simulink model "BLDC_SVM"  (R2023b)
settings: Solver=FixedStepDiscrete  StartTime=0.0  StopTime=10  FixedStep=1e-5  RelTol=1e-5
undefined symbols (not defined in the file): DiscIntNeverNeededParam
libraries: slpidlib x3, simulink x3, spsCurrentMeasurementLib x2, spsAlphaBetaZerotodq0Lib x1, spsDCVoltageSourceLib x1, spsPermanentMagnetSynchronousMachineLib x1, spsSVPWMGenerator2LevelLib x1, spsUniversalBridgeLib x1, spsVoltageMeasurementLib x1, spsabctoAlphaBetaZeroLib x1, spsdq0toAlphaBetaZeroLib x1, sps_lib x1
settings Model: Creator=84339  LastModifiedBy=84339
settings OptimizationCC: DefaultParameterBehavior=Inlined  EnhancedBackFolding=on  PassReuseOutputArgsAs=Individual arguments  ZeroExternalMemoryAtStartup=off  ZeroInternalMemoryAtStartup=off  OptimizeBlockOrder=speed  DifferentSizesBufferReuse=on  OptimizationCustomize=off  EfficientTunableParamExpr=on
settings DebuggingCC: ParameterTunabilityLossMsg=error
settings SFSimCC: MATLABDynamicMemAlloc=off
settings RTWCC: Description=Embedded Coder  SystemTargetFile=ert.tlc  GenCodeOnly=on  TemplateMakefile=ert_default_tmf
settings CodeAppCC: ForceParamTrailComments=on  IgnoreCustomStorageClasses=off  OperatorAnnotations=on  SimulinkDataObjDesc=on  SFDataObjDesc=on  InsertBlockDesc=on
settings ERTTargetCC: TargetLangStandard=C99 (ISO)  GenerateSampleERTMain=on  SupportContinuousTime=on  InlinedParameterPlacement=NonHierarchical  ERTCustomFileTemplate=example_file_process.tlc

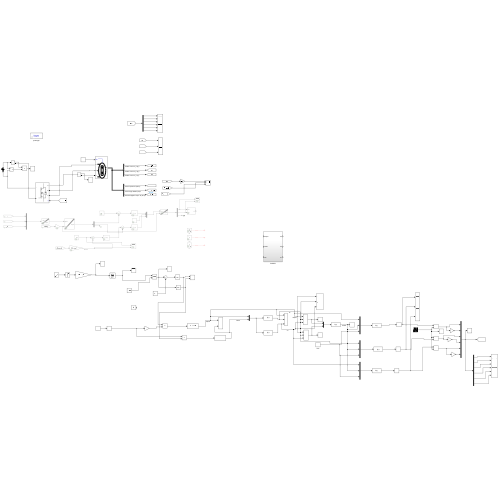
[thumbnail: Simulink's stored preview of the top-level diagram]
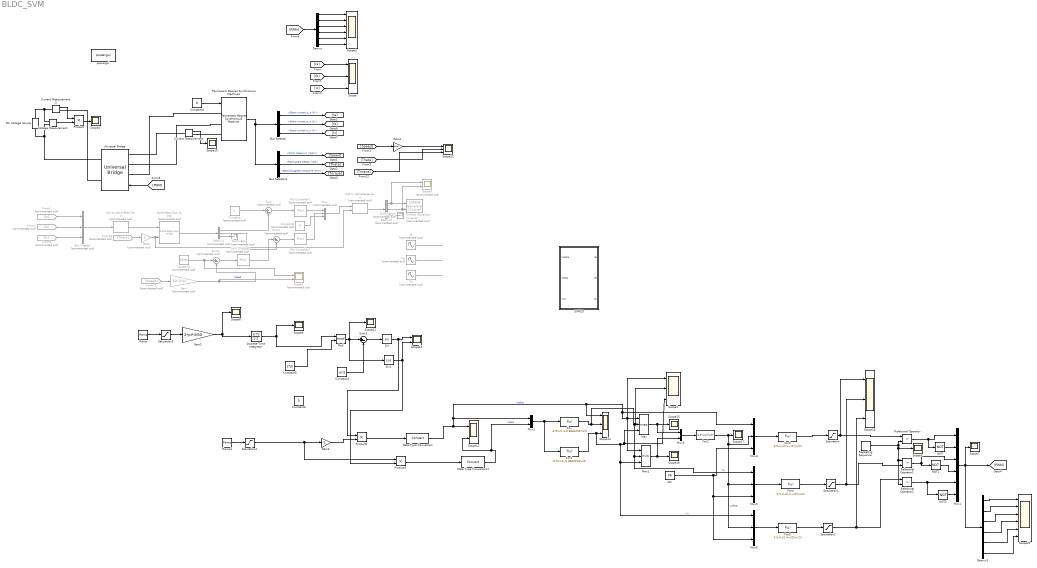
== system BLDC_SVM ==
  Alpha-Beta-Zero to dq0 : spsAlphaBetaZerotodq0Lib/Alpha-Beta-Zero to dq0  Commented=on  Alignment=90 degrees behind phase A axis
  Bus Creator : BusCreator  Commented=on  Inputs=3
  Bus Selector : BusSelector  OutputSignals=Stator current is_a (A),Stator current is_b (A),Stator current is_c (A)
  Bus Selector1 : BusSelector  OutputSignals=Rotor speed wm (rad/s),Rotor angle thetam (rad),Electromagnetic torque Te (N*m)
  Constant : Constant  Commented=on  Value=0
  Constant1 : Constant  Commented=on  Value=2500
  Constant2 : Constant  Commented=on  Value=0
  Constant3 : Constant  Value=pi/2  OutDataTypeStr=single
  Constant4 : Constant  Value=0
  Constant5 : Constant  Value=2*pi  OutDataTypeStr=single
  Constant6 : Constant  Value=0
  Current Measurement : spsCurrentMeasurementLib/Current Measurement  PhasorSimulation=off  OutputType=Complex  PSBequivalent=0
  Current Measurement3 : spsCurrentMeasurementLib/Current Measurement  PhasorSimulation=off  OutputType=Complex  PSBequivalent=0
  DC Voltage Source : spsDCVoltageSourceLib/DC Voltage Source  Amplitude=36  Measurements=None
  Data Type Conversion : DataTypeConversion  SaturateOnIntegerOverflow=off  RndMeth=Floor
  Data Type Conversion1 : DataTypeConversion  SaturateOnIntegerOverflow=off  RndMeth=Floor
  Demux : Demux  Outputs=6
  Demux1 : Demux  Commented=on  Outputs=3
  Demux2 : Demux  Commented=on  Outputs=3
  Demux3 : Demux  Outputs=6
  Discrete-Time Integrator : DiscreteIntegrator  SampleTime=1e-4  ICPrevOutput=DiscIntNeverNeededParam  ICPrevScaledInput=DiscIntNeverNeededParam
  Fcn : Fcn  Expr=-0.5*u(1)+0.8660254*u(2)
  Fcn1 : Fcn  Expr=-0.5*u(1)-0.8660254*u(2)
  Fcn2 : Fcn  Expr=-0.5*(u(1)+u(2))
  Fcn3 : Fcn  Expr=0.5+(u(1)+u(2))/u(3)
  Fcn4 : Fcn  Expr=0.5+(u(1)+u(2))/u(3)
  Fcn5 : Fcn  Expr=0.5+(u(1)+u(2))/u(3)
  From10 : From  Commented=on  GotoTag=Theta
  From11 : From  Commented=on  GotoTag=Speed
  From6 : From  Commented=on  GotoTag=Ia
  From7 : From  Commented=on  GotoTag=Ib
  From8 : From  Commented=on  GotoTag=Ic
  Gain : Gain  Commented=on  Gain=60/(2*pi)
  Gain1 : Gain  Commented=on  Gain=4
  Gain2 : Gain  Gain=2*pi*4/60  OutDataTypeStr=single
  Gain3 : Gain  Gain=-1
  Gain4 : Gain  Gain=30/pi
  Max : MinMax  Function=max  Inputs=3
  Max1 : MinMax  Inputs=3
  Mod : Math  Operator=mod
  Mux : Mux  Commented=on  Inputs=3
  Mux1 : Mux  Inputs=6
  Mux2 : Mux  Inputs=2
  Mux3 : Mux  Inputs=2
  Mux4 : Mux  Inputs=3
  Mux5 : Mux  Inputs=3
  Mux6 : Mux  Inputs=3
  NOT : Logic  Operator=NOT  IconShape=distinctive  AllPortsSameDT=off  OutDataTypeStr=boolean
  NOT1 : Logic  Operator=NOT  IconShape=distinctive  AllPortsSameDT=off  OutDataTypeStr=boolean
  NOT2 : Logic  Operator=NOT  IconShape=distinctive  AllPortsSameDT=off  OutDataTypeStr=boolean
  PID Controller : slpidlib/PID Controller  Commented=on  Controller=PI  Form=Parallel  TimeDomain=Discrete-time  UseExternalTs=off  SampleTime=1e-5  IntegratorMethod=Forward Euler  FilterMethod=Forward Euler  ControllerParametersSource=internal  P=0.1  I=0.01  UseKiTs=off  D=0  N=100  UseFilter=on  TunerSelectOption=Transfer Function Based (PID Tuner App)  InitialConditionSource=internal  InitialConditionForIntegrator=0  InitialConditionForFilter=0  DifferentiatorICPrevScaledInput=0  ExternalReset=none  TrackingMode=off  Kt=1  LimitOutput=off  SatLimitsSource=internal  UpperSaturationLimit=inf  LowerSaturationLimit=-inf  LinearizeAsGain=on  AntiWindupMode=none  Kb=1  LimitIntegrator=off  UpperIntegratorSaturationLimit=inf  LowerIntegratorSaturationLimit=-inf  POutMin=[]  POutMax=[]  IOutMin=[]  IOutMax=[]  DOutMin=[]  DOutMax=[]  NOutMin=[]  NOutMax=[]  SumOutMin=[]  SumOutMax=[]  SaturationOutMin=[]  SaturationOutMax=[]  PParamMin=[]  PParamMax=[]  IParamMin=[]  IParamMax=[]  DParamMin=[]  DParamMax=[]  NParamMin=[]  NParamMax=[]  KbParamMin=[]  KbParamMax=[]  KtParamMin=[]  KtParamMax=[]  KbOutMin=[]  KbOutMax=[]  KtOutMin=[]  KtOutMax=[]  IntegratorOutMin=[]  IntegratorOutMax=[]  FilterOutMin=[]  FilterOutMax=[]  SumI1OutMin=[]  SumI1OutMax=[]  SumI2OutMin=[]  SumI2OutMax=[]  SumI3OutMin=[]  SumI3OutMax=[]  SumI4OutMin=[]  SumI4OutMax=[]  SumDOutMin=[]  SumDOutMax=[]  DifferentiatorOutMin=[]  DifferentiatorOutMax=[]  FilterDiffOutCoefMin=[]  FilterDiffOutCoefMax=[]  ReciprocalOutMin=[]  ReciprocalOutMax=[]  SumDenOutMin=[]  SumDenOutMax=[]  SumNumOutMin=[]  SumNumOutMax=[]  DivideOutMin=[]  DivideOutMax=[]  UdiffTsProdOutMin=[]  UdiffTsProdOutMax=[]  NTsProdOutMin=[]  NTsProdOutMax=[]  UintegralTsProdOutMin=[]  UintegralTsProdOutMax=[]  UngainTsProdOutMin=[]  UngainTsProdOutMax=[]  ClampingZeroOutDataTypeStr=Inherit: Inherit via back propagation  ClampingZeroOutMin=[]  ClampingZeroOutMax=[]  FilterDenConstantOutDataTypeStr=Inherit: Inherit via back propagation  FilterDenConstantOutMin=[]  FilterDenConstantOutMax=[]  PCopyOutDataTypeStr=Inherit: Inherit via back propagation  PCopyOutMin=[]  PCopyOutMax=[]  NCopyOutDataTypeStr=Inherit: Inherit via back propagation  NCopyOutMin=[]  NCopyOutMax=[]  IntegratorContinuousStateAttributes=''  IntegratorStateMustResolveToSignalObject=off  IntegratorRTWStateStorageClass=Auto  FilterContinuousStateAttributes=''  FilterStateMustResolveToSignalObject=off  FilterRTWStateStorageClass=Auto  ParallelPVariant=InternalParameters  IdealPVariant=Disabled  IVariant=InternalParameters  DVariant=Disabled  IntegratorVariant=Discrete  SatVariant=Disabled  AWVariant=Passthrough  PCopyVariant=Disabled  TRVariant=Disabled  FdbkBlocksVariant=Forward  IdealPFdbkVariant=Disabled  SatFdbkVariant=Disabled  DerivativeFilterVariant=Disabled  NVariant=Disabled  NCopyVariant=Disabled_SignalSpec  FilterICVariant=Disabled  IntegratorICVariant=InternalICs  ExternalResetVariant=Disabled  TRSumVariant=Passthrough  SumFdbkVariant=Disabled  SumVariant=Sum_PI  TsampFilterVariant=InternalTs  TsampNgainVariant=Passthrough  TsampIntegralVariant=Disabled_SignalSpec  ExternalSaturationOutDataTypeStr=Inherit: Same as second input
  PID Controller1 : slpidlib/PID Controller  Commented=on  Controller=PI  Form=Parallel  TimeDomain=Discrete-time  UseExternalTs=off  SampleTime=1e-5  IntegratorMethod=Forward Euler  FilterMethod=Forward Euler  ControllerParametersSource=internal  P=1  I=0.01  UseKiTs=off  D=0  N=100  UseFilter=on  TunerSelectOption=Transfer Function Based (PID Tuner App)  InitialConditionSource=internal  InitialConditionForIntegrator=0  InitialConditionForFilter=0  DifferentiatorICPrevScaledInput=0  ExternalReset=none  TrackingMode=off  Kt=1  LimitOutput=off  SatLimitsSource=internal  UpperSaturationLimit=inf  LowerSaturationLimit=-inf  LinearizeAsGain=on  AntiWindupMode=none  Kb=1  LimitIntegrator=off  UpperIntegratorSaturationLimit=inf  LowerIntegratorSaturationLimit=-inf  POutMin=[]  POutMax=[]  IOutMin=[]  IOutMax=[]  DOutMin=[]  DOutMax=[]  NOutMin=[]  NOutMax=[]  SumOutMin=[]  SumOutMax=[]  SaturationOutMin=[]  SaturationOutMax=[]  PParamMin=[]  PParamMax=[]  IParamMin=[]  IParamMax=[]  DParamMin=[]  DParamMax=[]  NParamMin=[]  NParamMax=[]  KbParamMin=[]  KbParamMax=[]  KtParamMin=[]  KtParamMax=[]  KbOutMin=[]  KbOutMax=[]  KtOutMin=[]  KtOutMax=[]  IntegratorOutMin=[]  IntegratorOutMax=[]  FilterOutMin=[]  FilterOutMax=[]  SumI1OutMin=[]  SumI1OutMax=[]  SumI2OutMin=[]  SumI2OutMax=[]  SumI3OutMin=[]  SumI3OutMax=[]  SumI4OutMin=[]  SumI4OutMax=[]  SumDOutMin=[]  SumDOutMax=[]  DifferentiatorOutMin=[]  DifferentiatorOutMax=[]  FilterDiffOutCoefMin=[]  FilterDiffOutCoefMax=[]  ReciprocalOutMin=[]  ReciprocalOutMax=[]  SumDenOutMin=[]  SumDenOutMax=[]  SumNumOutMin=[]  SumNumOutMax=[]  DivideOutMin=[]  DivideOutMax=[]  UdiffTsProdOutMin=[]  UdiffTsProdOutMax=[]  NTsProdOutMin=[]  NTsProdOutMax=[]  UintegralTsProdOutMin=[]  UintegralTsProdOutMax=[]  UngainTsProdOutMin=[]  UngainTsProdOutMax=[]  ClampingZeroOutDataTypeStr=Inherit: Inherit via back propagation  ClampingZeroOutMin=[]  ClampingZeroOutMax=[]  FilterDenConstantOutDataTypeStr=Inherit: Inherit via back propagation  FilterDenConstantOutMin=[]  FilterDenConstantOutMax=[]  PCopyOutDataTypeStr=Inherit: Inherit via back propagation  PCopyOutMin=[]  PCopyOutMax=[]  NCopyOutDataTypeStr=Inherit: Inherit via back propagation  NCopyOutMin=[]  NCopyOutMax=[]  IntegratorContinuousStateAttributes=''  IntegratorStateMustResolveToSignalObject=off  IntegratorRTWStateStorageClass=Auto  FilterContinuousStateAttributes=''  FilterStateMustResolveToSignalObject=off  FilterRTWStateStorageClass=Auto  ParallelPVariant=InternalParameters  IdealPVariant=Disabled  IVariant=InternalParameters  DVariant=Disabled  IntegratorVariant=Discrete  SatVariant=Disabled  AWVariant=Passthrough  PCopyVariant=Disabled  TRVariant=Disabled  FdbkBlocksVariant=Forward  IdealPFdbkVariant=Disabled  SatFdbkVariant=Disabled  DerivativeFilterVariant=Disabled  NVariant=Disabled  NCopyVariant=Disabled_SignalSpec  FilterICVariant=Disabled  IntegratorICVariant=InternalICs  ExternalResetVariant=Disabled  TRSumVariant=Passthrough  SumFdbkVariant=Disabled  SumVariant=Sum_PI  TsampFilterVariant=InternalTs  TsampNgainVariant=Passthrough  TsampIntegralVariant=Disabled_SignalSpec  ExternalSaturationOutDataTypeStr=Inherit: Same as second input
  PID Controller2 : slpidlib/PID Controller  Commented=on  Controller=PI  Form=Parallel  TimeDomain=Discrete-time  UseExternalTs=off  SampleTime=1e-5  IntegratorMethod=Forward Euler  FilterMethod=Forward Euler  ControllerParametersSource=internal  P=1  I=0.01  UseKiTs=off  D=0  N=100  UseFilter=on  TunerSelectOption=Transfer Function Based (PID Tuner App)  InitialConditionSource=internal  InitialConditionForIntegrator=0  InitialConditionForFilter=0  DifferentiatorICPrevScaledInput=0  ExternalReset=none  TrackingMode=off  Kt=1  LimitOutput=off  SatLimitsSource=internal  UpperSaturationLimit=inf  LowerSaturationLimit=-inf  LinearizeAsGain=on  AntiWindupMode=none  Kb=1  LimitIntegrator=off  UpperIntegratorSaturationLimit=inf  LowerIntegratorSaturationLimit=-inf  POutMin=[]  POutMax=[]  IOutMin=[]  IOutMax=[]  DOutMin=[]  DOutMax=[]  NOutMin=[]  NOutMax=[]  SumOutMin=[]  SumOutMax=[]  SaturationOutMin=[]  SaturationOutMax=[]  PParamMin=[]  PParamMax=[]  IParamMin=[]  IParamMax=[]  DParamMin=[]  DParamMax=[]  NParamMin=[]  NParamMax=[]  KbParamMin=[]  KbParamMax=[]  KtParamMin=[]  KtParamMax=[]  KbOutMin=[]  KbOutMax=[]  KtOutMin=[]  KtOutMax=[]  IntegratorOutMin=[]  IntegratorOutMax=[]  FilterOutMin=[]  FilterOutMax=[]  SumI1OutMin=[]  SumI1OutMax=[]  SumI2OutMin=[]  SumI2OutMax=[]  SumI3OutMin=[]  SumI3OutMax=[]  SumI4OutMin=[]  SumI4OutMax=[]  SumDOutMin=[]  SumDOutMax=[]  DifferentiatorOutMin=[]  DifferentiatorOutMax=[]  FilterDiffOutCoefMin=[]  FilterDiffOutCoefMax=[]  ReciprocalOutMin=[]  ReciprocalOutMax=[]  SumDenOutMin=[]  SumDenOutMax=[]  SumNumOutMin=[]  SumNumOutMax=[]  DivideOutMin=[]  DivideOutMax=[]  UdiffTsProdOutMin=[]  UdiffTsProdOutMax=[]  NTsProdOutMin=[]  NTsProdOutMax=[]  UintegralTsProdOutMin=[]  UintegralTsProdOutMax=[]  UngainTsProdOutMin=[]  UngainTsProdOutMax=[]  ClampingZeroOutDataTypeStr=Inherit: Inherit via back propagation  ClampingZeroOutMin=[]  ClampingZeroOutMax=[]  FilterDenConstantOutDataTypeStr=Inherit: Inherit via back propagation  FilterDenConstantOutMin=[]  FilterDenConstantOutMax=[]  PCopyOutDataTypeStr=Inherit: Inherit via back propagation  PCopyOutMin=[]  PCopyOutMax=[]  NCopyOutDataTypeStr=Inherit: Inherit via back propagation  NCopyOutMin=[]  NCopyOutMax=[]  IntegratorContinuousStateAttributes=''  IntegratorStateMustResolveToSignalObject=off  IntegratorRTWStateStorageClass=Auto  FilterContinuousStateAttributes=''  FilterStateMustResolveToSignalObject=off  FilterRTWStateStorageClass=Auto  ParallelPVariant=InternalParameters  IdealPVariant=Disabled  IVariant=InternalParameters  DVariant=Disabled  IntegratorVariant=Discrete  SatVariant=Disabled  AWVariant=Passthrough  PCopyVariant=Disabled  TRVariant=Disabled  FdbkBlocksVariant=Forward  IdealPFdbkVariant=Disabled  SatFdbkVariant=Disabled  DerivativeFilterVariant=Disabled  NVariant=Disabled  NCopyVariant=Disabled_SignalSpec  FilterICVariant=Disabled  IntegratorICVariant=InternalICs  ExternalResetVariant=Disabled  TRSumVariant=Passthrough  SumFdbkVariant=Disabled  SumVariant=Sum_PI  TsampFilterVariant=InternalTs  TsampNgainVariant=Passthrough  TsampIntegralVariant=Disabled_SignalSpec  ExternalSaturationOutDataTypeStr=Inherit: Same as second input
  Permanent Magnet Synchronous Machine1 : spsPermanentMagnetSynchronousMachineLib/Permanent Magnet Synchronous Machine  NbPhases=3  FluxDistribution=Trapezoidal  RotorType=Round  MechanicalLoad=Torque Tm  PresetModel=No  ShowDetailedParameters=on  MeasurementBus=off  Resistance=0.0485  Inductance=8.5e-3  dqInductances=[8.5e-3,8.5e-3]  La=0.000395  MachineConstant=Flux linkage established by magnets (V.s)  Flux=0.1194  VoltageCst=100.0283  TorqueCst=0.9552  Flat=120  Mechanical=[0.0027 0.0004924 4 0]  PolePairs=4  InitialConditions=[0,0, 0,0]  InitialConditions5ph=[0 0 0 0 0 0]  RefAngle=90 degrees behind phase A axis (modified Park)  IterativeDiscreteModel=Trapezoidal non iterative  TsBlock=-1  TsPowergui=0
  Product : Product
  Product2 : Product
  Product3 : Product
  Ramp : simulink/Sources/Ramp  slope=100  start=0  InitialOutput=0
  Ramp1 : simulink/Sources/Ramp  slope=100  start=0  InitialOutput=0
  Relational Operator : RelationalOperator  Operator=>  OutDataTypeStr=boolean  RndMeth=Simplest  InputSameDT=off
  Relational Operator1 : RelationalOperator  Operator=>  OutDataTypeStr=boolean  RndMeth=Simplest  InputSameDT=off
  Relational Operator2 : RelationalOperator  Operator=>  OutDataTypeStr=boolean  RndMeth=Simplest  InputSameDT=off
  Repeating Sequence : simulink/Sources/Repeating Sequence  rep_seq_t=[0 1/10000]  rep_seq_y=[0 1]
  SVM2D : Subsystem
  SVPWM Generator (2-Level) : spsSVPWMGenerator2LevelLib/SVPWM Generator (2-Level)  Commented=on  InputType=alpha-beta components  SwitchingPattern=Pattern #1  Fc=10000  ParUref=[0.8 -30 50]  Ts=1e-5
  Saturation : Saturate  UpperLimit=1  LowerLimit=0
  Saturation1 : Saturate  UpperLimit=1  LowerLimit=0
  Saturation2 : Saturate  UpperLimit=1  LowerLimit=0
  Saturation3 : Saturate  UpperLimit=300  LowerLimit=0
  Saturation4 : Saturate  UpperLimit=6  LowerLimit=0
  Scope{,1,12,14,18} (5 alike) : Scope  NumInputPorts=3
  Scope10 : Scope  NumInputPorts=2
  Scope{4,6..9,11,15..17,19} (10 alike) : Scope
  Scope13 : Scope  NumInputPorts=2
  Scope2 : Scope  Commented=on  NumInputPorts=2
  Scope20 : Scope  NumInputPorts=6
  Scope3 : Scope  NumInputPorts=6
  Scope5 : Scope  Commented=on  NumInputPorts=2
  Sin : Trigonometry
  Sin1 : Trigonometry  Operator=cos
  Sum : Sum  Commented=on  Inputs=|+-
  Sum1 : Sum  Commented=on  Inputs=|+-
  Sum2 : Sum  Commented=on  Inputs=|+-
  Sum3 : Sum  Inputs=|+-
  Terminator : Terminator  Commented=on
  Terminator1 : Terminator  Commented=on
  Universal Bridge : spsUniversalBridgeLib/Universal Bridge  Arms=3  SnubberResistance=1e5  SnubberCapacitance=inf  Device=MOSFET / Diodes  Ron=1e-3  Lon=0  ForwardVoltages="[  0  0  ]"  ForwardVoltage=0  GTOparameters=[ 10e-6 , 20e-6 ]  IGBTparameters=[ 1e-6 , 2e-6 ]  Measurements=None  Measurements_2=None  converterType=Rectifier
  Va : Sin  Commented=on  Amplitude=14*sqrt(2)  Frequency=100*pi  SampleTime=1e-5
  Vb : Sin  Commented=on  Amplitude=14*sqrt(2)  Frequency=100*pi  Phase=-2*pi/3  SampleTime=1e-5
  Vc : Sin  Commented=on  Amplitude=14*sqrt(2)  Frequency=100*pi  Phase=2*pi/3  SampleTime=1e-5
  Vdc : Constant  Value=36  OutDataTypeStr=single
  Voltage Measurement : spsVoltageMeasurementLib/Voltage Measurement  PhasorSimulation=off  OutputType=Complex  PSBequivalent=0
  abc to Alpha-Beta-Zero : spsabctoAlphaBetaZeroLib/abc to Alpha-Beta-Zero  Commented=on
  dq0 to Alpha-Beta-Zero : spsdq0toAlphaBetaZeroLib/dq0 to Alpha-Beta-Zero  Commented=on  Alignment=90 degrees behind phase A axis
  powergui : sps_lib/powergui  Priority=1  SimulationMode=Discrete  SampleTime=1e-5  frequency=60  Iterations=50  frequencyindice=0  Pbase=100e6  ErrMax=1e-4  UnitsV=kV  UnitsW=MW  buscounter=0  FunctionMessages=off  echomessages=off  EnableUseOfTLC=off  CurrentSourceSwitches=off  DisableSnubberDevices=off  DisableRonSwitches=off  DisableVfSwitches=off  DisplayEquations=off  AutomaticDiscreteSolvers=off  SolverType=Tustin/Backward Euler (TBE)  Interpol=off  ExternalGateDelay=off  methode=off  Ts=100  x0status=blocks  SPID=on  SwTol=0  HookPort=off  NonlinearTolerance=1e-4  nMaxIteration=100  ContinueOnMaxIteration=off  RestoreLinks=warning  ResistiveCurrentMeasurement=off  Frange=[0:2:500]  Ylog=off  Xlog=on  ShowGrid=off  save=off  variable=ZData  structure=0  ZoomFFT=off  StartTime=0.0  cycles=1  DisplayStyle=1  fundamental=60  FreqAxis=off  MaxFrequency=1000  frequencyindicesteady=1  RmsSteady=1  display=off
  wires:
  Permanent Magnet Synchronous Machine1/1 -> Bus Selector1/1, Bus Selector/1
  [Ia] -> Scope/1
  [Ib] -> Scope/2
  [Ic] -> Scope/3
  [PWM] -> Demux/1
  Demux/1 -> Scope3/1
  Demux/2 -> Scope3/2
  Demux/3 -> Scope3/3
  Demux/4 -> Scope3/4
  Demux/5 -> Scope3/5
  Demux/6 -> Scope3/6
  Current Measurement3/1 -> Product/1
  Voltage Measurement/1 -> Product/2
  Product/1 -> Scope4/1
  Bus Selector/1 -> [Ia]  "<Stator current is_a (A)>"
  Bus Selector/2 -> [Ib]  "<Stator current is_b (A)>"
  Bus Selector/3 -> [Ic]  "<Stator current is_c (A)>"
  From6/1 -> Bus Creator/1
  From7/1 -> Bus Creator/2
  From8/1 -> Bus Creator/3
  Bus Creator/1 -> abc to Alpha-Beta-Zero/1
  abc to Alpha-Beta-Zero/1 -> Alpha-Beta-Zero to dq0/1
  Bus Selector1/1 -> [Speed]  "<Rotor speed wm (rad/s)>"
  Bus Selector1/2 -> [Theta]  "<Rotor angle thetam (rad)>"
  From10/1 -> Gain1/1
  [PWM] -> Universal Bridge/1
  Bus Selector1/3 -> [Torque]  "<Electromagnetic torque Te (N*m)>"
  Gain1/1 -> dq0 to Alpha-Beta-Zero/2, Alpha-Beta-Zero to dq0/2
  From11/1 -> Gain/1
  Alpha-Beta-Zero to dq0/1 -> Demux1/1
  Demux1/1 -> Sum/2
  Demux1/2 -> Sum1/2
  Constant/1 -> Sum/1
  Sum2/1 -> PID Controller/1
  Gain/1 -> Scope2/2, Sum2/2  "Speed"
  Constant1/1 -> Scope2/1, Sum2/1
  PID Controller/1 -> Sum1/1
  Sum/1 -> PID Controller1/1
  Sum1/1 -> PID Controller2/1
  Demux1/3 -> Terminator/1
  PID Controller1/1 -> Mux/1
  Mux/1 -> dq0 to Alpha-Beta-Zero/1
  PID Controller2/1 -> Mux/2
  Constant2/1 -> Mux/3
  dq0 to Alpha-Beta-Zero/1 -> Demux2/1
  Demux2/3 -> Terminator1/1
  Demux2/1 -> Scope5/1, SVPWM Generator (2-Level)/1
  Demux2/2 -> Scope5/2, SVPWM Generator (2-Level)/2
  NOT/1 -> Mux1/2
  NOT1/1 -> Mux1/4
  NOT2/1 -> Mux1/6
  Mux1/1 -> Demux3/1, Scope7/1, [PWM]
  Repeating Sequence/1 -> Relational Operator2/2, Relational Operator1/1, Scope6/1, Relational Operator/2
  Saturation/1 -> Scope18/1, Relational Operator/1
  Relational Operator/1 -> NOT/1, Mux1/1
  Saturation1/1 -> Scope18/2, Relational Operator1/2
  Relational Operator1/1 -> Mux1/3, NOT1/1
  Saturation2/1 -> Scope18/3, Relational Operator2/1
  Relational Operator2/1 -> NOT2/1, Mux1/5
  Ramp/1 -> Saturation3/1
  Va/1 -> ?
  Vc/1 -> ?
  Vb/1 -> ?
  Constant5/1 -> Mod/2
  Gain2/1 -> Scope8/1, Discrete-Time Integrator/1
  Discrete-Time Integrator/1 -> Mod/1, Scope9/1
  Mod/1 -> Sum3/1, Sin1/1, Scope11/1
  Sin/1 -> Product2/1, Scope10/1
  Sin1/1 -> Product3/2, Scope10/2
  Saturation4/1 -> Product3/1, Gain3/1
  Gain3/1 -> Product2/2
  Product2/1 -> Data Type Conversion/1
  Product3/1 -> Data Type Conversion1/1
  [Speed] -> Gain4/1
  Data Type Conversion1/1 -> Scope13/2, Mux2/2  "Vbeta"
  Mux2/1 -> Fcn1/1, Fcn/1
  Fcn/1 -> Mux5/1, Max1/2, Scope1/2, Max/2, Scope14/2  "Vb"
  Fcn1/1 -> Max1/3, Mux6/1, Scope1/3, Max/3, Scope14/3  "Vc"
  Max/1 -> Mux3/1, Scope15/1
  Data Type Conversion/1 -> Scope14/1, Mux4/1, Max1/1, Scope1/1, Max/1, Mux2/1, Scope13/1  "Valpha"
  Max1/1 -> Mux3/2, Scope16/1
  Mux3/1 -> Fcn2/1
  Fcn2/1 -> Mux6/2, Mux5/2, Mux4/2, Scope17/1  "Voffset"
  Vdc/1 -> Mux6/3, Mux5/3, Mux4/3
  Mux4/1 -> Fcn3/1
  Mux5/1 -> Fcn4/1
  Mux6/1 -> Fcn5/1
  Fcn3/1 -> Saturation/1
  Fcn4/1 -> Saturation1/1
  Fcn5/1 -> Saturation2/1
  Constant4/1 -> Permanent Magnet Synchronous Machine1/1
  Demux3/1 -> Scope20/1
  Demux3/2 -> Scope20/2
  Demux3/3 -> Scope20/3
  Demux3/4 -> Scope20/4
  Demux3/5 -> Scope20/5
  Demux3/6 -> Scope20/6
  Gain4/1 -> Scope12/1
  Saturation3/1 -> Gain2/1
  Ramp1/1 -> Saturation4/1
  [Theta] -> Scope12/2
  [Torque] -> Scope12/3
  Constant3/1 -> Sum3/2
  Sum3/1 -> Sin/1
  Current Measurement/1 -> Scope19/1
  connections:
  DC Voltage Source/LConn1 -- Universal Bridge/RConn2 -- Voltage Measurement/LConn2
  Current Measurement3/LConn1 -- DC Voltage Source/RConn1 -- Voltage Measurement/LConn1
  Universal Bridge/RConn1 -- Current Measurement3/RConn1
  Universal Bridge/LConn1 -- Permanent Magnet Synchronous Machine1/LConn1
  Universal Bridge/LConn2 -- Permanent Magnet Synchronous Machine1/LConn2
  Current Measurement/LConn1 -- Universal Bridge/LConn3
  Current Measurement/RConn1 -- Permanent Magnet Synchronous Machine1/LConn3

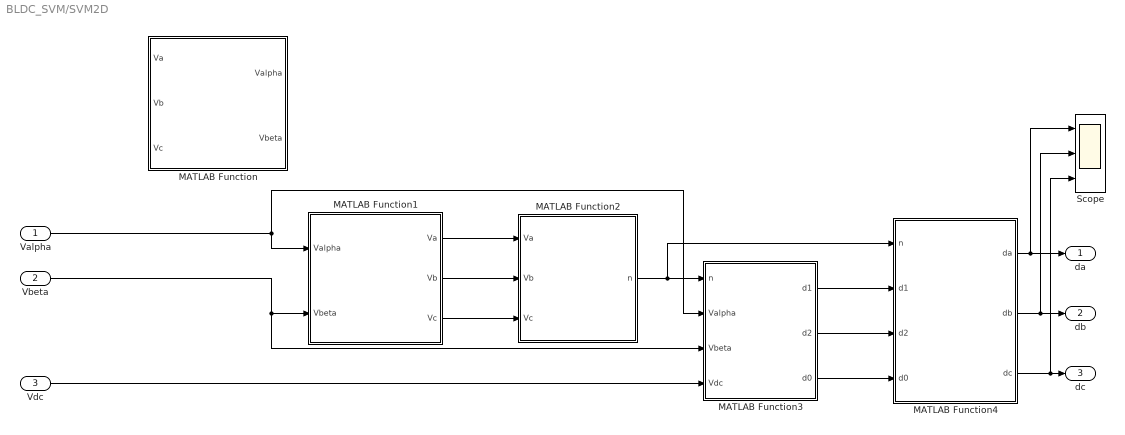
== system BLDC_SVM/SVM2D ==
  Valpha : Inport
  Vbeta : Inport  Port=2
  Vdc : Inport  Port=3
  MATLAB Function : MATLAB Function  TreatAsAtomicUnit=on
  MATLAB Function1 : MATLAB Function  TreatAsAtomicUnit=on
  MATLAB Function2 : MATLAB Function  TreatAsAtomicUnit=on
  MATLAB Function3 : MATLAB Function  TreatAsAtomicUnit=on
  MATLAB Function4 : MATLAB Function  TreatAsAtomicUnit=on
  Scope : Scope  NumInputPorts=3
  da : Outport
  db : Outport  Port=2
  dc : Outport  Port=3
  wires:
  MATLAB Function3/1(d1) -> MATLAB Function4/2(d1)
  MATLAB Function1/1(Va) -> MATLAB Function2/1(Va)
  Vdc/1 -> MATLAB Function3/4(Vdc)
  MATLAB Function4/2(db) -> Scope/2, db/1
  Vbeta/1 -> MATLAB Function3/3(Vbeta), MATLAB Function1/2(Vbeta)
  MATLAB Function3/2(d2) -> MATLAB Function4/3(d2)
  MATLAB Function2/1(n) -> MATLAB Function4/1(n), MATLAB Function3/1(n)
  MATLAB Function1/3(Vc) -> MATLAB Function2/3(Vc)
  MATLAB Function1/2(Vb) -> MATLAB Function2/2(Vb)
  MATLAB Function3/3(d0) -> MATLAB Function4/4(d0)
  Valpha/1 -> MATLAB Function1/1(Valpha), MATLAB Function3/2(Valpha)
  MATLAB Function4/1(da) -> Scope/1, da/1
  MATLAB Function4/3(dc) -> Scope/3, dc/1

== matlab function BLDC_SVM/SVM2D/MATLAB Function1 ==
  data: Valpha input single; Va output single; Vbeta input single; Vb output single; Vc output single
function [Va,Vb,Vc] = Rev_Clark(Valpha,Vbeta)
Va = Valpha;
Vb = -Valpha/2 + sqrt(3)*Vbeta/2;
Vc = -Valpha/2 - sqrt(3)*Vbeta/2;

== matlab function BLDC_SVM/SVM2D/MATLAB Function ==
  data: Va input single; Valpha output single; Vb input single; Vc input single; Vbeta output single
function [Valpha,Vbeta] = Clark(Va,Vb,Vc)
Valpha = 2/3*(Va-Vb/2-Vc/2);
Vbeta = 2/3*sqrt(3)/2*(Vb-Vc);

== matlab function BLDC_SVM/SVM2D/MATLAB Function2 ==
  data: Va input single; n output single; Vb input single; Vc input single
function n = Sector(Va,Vb,Vc)
n = single(0);
if (Va >= Vb)
    if(Vb >= Vc)
        n = single(1);
    else
        if (Vc >= Va)
            n = single(5);
        else
            n = single(6);
        end
    end
else
    if (Vb < Vc)
        n = single(4);
    else
        if (Vc < Va)
            n = single(2);
        else
            n = single(3);
        end
    end
end

== matlab function BLDC_SVM/SVM2D/MATLAB Function3 ==
  data: n input single; Valpha input single; Vbeta input single; d1 output single; Vdc input single; d2 output single; d0 output single
function [d1,d2,d0] = Duty(n,Valpha,Vbeta,Vdc)
d0 = single(0);
d1 = single(0);
d2 = single(0);
if (n == 1)
    d1 = 1/Vdc*(3/2*Valpha - sqrt(3)/2*Vbeta);
    d2 = 1/Vdc*(0*Valpha + sqrt(3)*Vbeta);
    d0 = 1-d1-d2;
end
if (n == 2)
    d1 = 1/Vdc*(-3/2*Valpha + sqrt(3)/2*Vbeta);
    d2 = 1/Vdc*(3/2*Valpha + sqrt(3)/2*Vbeta);
    d0 = 1-d1-d2;
end
if (n == 3)
    d1 = 1/Vdc*(0*Valpha + sqrt(3)*Vbeta);
    d2 = 1/Vdc*(-3/2*Valpha - sqrt(3)/2*Vbeta);
    d0 = 1-d1-d2;
end
if (n == 4)
    d1 = 1/Vdc*(0*Valpha - sqrt(3)*Vbeta);
    d2 = 1/Vdc*(-3/2*Valpha + sqrt(3)/2*Vbeta);
    d0 = 1-d1-d2; 
end
if (n == 5)
    d1 = 1/Vdc*(-3/2*Valpha - sqrt(3)/2*Vbeta);
    d2 = 1/Vdc*(3/2*Valpha - sqrt(3)/2*Vbeta);
    d0 = 1-d1-d2;
end
if (n == 6)
    d1 = 1/Vdc*(3/2*Valpha + sqrt(3)/2*Vbeta);
    d2 = 1/Vdc*(0*Valpha - sqrt(3)*Vbeta);
    d0 = 1-d1-d2; 
end

== matlab function BLDC_SVM/SVM2D/MATLAB Function4 ==
  data: n input single; da output single; d1 input single; d2 input single; d0 input single; db output single; dc output single
function [da,db,dc] = Duty_Cycle(n,d1,d2,d0)
da = single(0);
db = single(0);
dc = single(0);
if (n == 1)
    da = d0/2;
    db = d0/2 + d1;
    dc = d0/2 + d1 + d2;
end
if (n == 2)
    da = d0/2 + d1;
    db = d0/2;
    dc = d0/2 + d1 + d2;
end
if (n == 3)
    da = d0/2 + d1 + d2;
    db = d0/2;
    dc = d0/2 + d1;
end
if (n == 4)
    da = d0/2 + d1 + d2;
    db = d0/2 + d1;
    dc = d0/2;
end
if (n == 5)
    da = d0/2 + d1;
    db = d0/2 + d1 + d2;
    dc = d0/2;
end
if (n == 6)
    da = d0/2;
    db = d0/2 + d1 + d2;
    dc = d0/2 + d1;
end
